simulink model "EDF"  (R2025b)
settings: Solver=VariableStepAuto  StartTime=0.0  StopTime=30  FixedStep=0.1  RelTol=1e-3
libraries: simulink x1, slpidlib x1
settings Model: Creator=wangzerun  LastModifiedBy=wangzerun

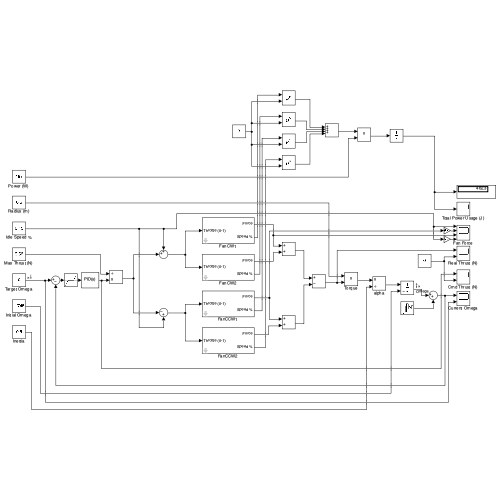
[thumbnail: Simulink's stored preview of the top-level diagram]
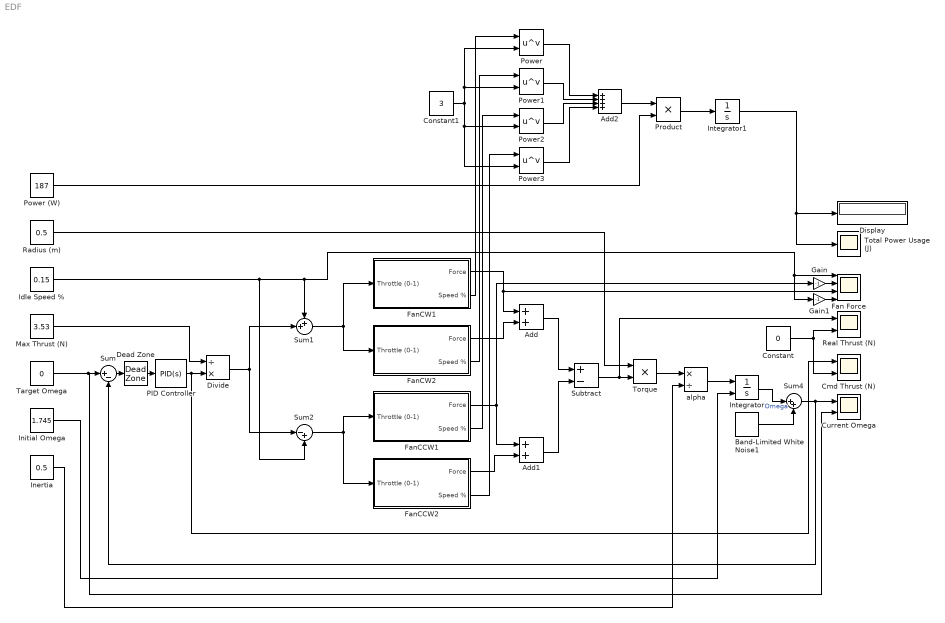
== system EDF ==
  Add : Sum
  Add1 : Sum
  Add2 : Sum  Inputs=++++
  Band-Limited White Noise1 : simulink/Sources/Band-Limited White Noise  Cov=(30 * pi/180)^2 * 2  Ts=2  seed=[23341]
  Cmd Thrust (N) : Scope  NumInputPorts=2
      settings: ActiveDisplayYMinimum=-12.321116744675173  ActiveDisplayYMaximum=4.742010611975001  DataLoggingVariableName=ScopeData3
  Constant : Constant  Value=0
  Constant1 : Constant  Value=3
  Current Omega : Scope  NumInputPorts=2
      settings: ActiveDisplayYMinimum=-4.3264371148966774  ActiveDisplayYMaximum=4.7874283495115693
  Dead Zone : DeadZone  LowerValue=-0.015  UpperValue=0.015
  Display : Display
  Divide : Product  Inputs=/*
  Fan Force : Scope  NumInputPorts=4
      settings: ActiveDisplayYMinimum=-5.5903004683370039  ActiveDisplayYMaximum=5.6346908697833626  DataLoggingVariableName=ScopeData4
  FanCCW1 : Subsystem  mask{tau=0.1, F_max=3.53}
      mask prompts: tau "Time Constant (s)"; F_max "Max Thrust (N)"
  FanCCW2 : Subsystem  mask{tau=0.15, F_max=3.53}
      mask prompts: tau "Time Constant (s)"; F_max "Max Thrust (N)"
  FanCW1 : Subsystem  mask{tau=0.1, F_max=3.53}
      mask prompts: tau "Time Constant (s)"; F_max "Max Thrust (N)"
  FanCW2 : Subsystem  mask{tau=0.1, F_max=3.53}
      mask prompts: tau "Time Constant (s)"; F_max "Max Thrust (N)"
  Gain : Gain  Gain=-1
  Gain1 : Gain  Gain=-1
  Idle Speed % : Constant  Value=0.15
  Inertia : Constant  Value=0.5
  Initial Omega : Constant  Value=1.745
  Integrator : Integrator  InitialConditionSource=external  InitialCondition=10
  Integrator1 : Integrator
  Max Thrust (N) : Constant  Value=3.53
  PID Controller : slpidlib/PID Controller  Controller=PID  Form=Parallel  TimeDomain=Continuous-time  UseExternalTs=off  SampleTime=0.1  IntegratorMethod=Forward Euler  FilterMethod=Forward Euler  ControllerParametersSource=internal  P=2.5  I=1  UseKiTs=off  D=4  UseExternalDerivativeSource=off  N=2  UseFilter=on  TunerSelectOption=Transfer Function Based (PID Tuner App)  InitialConditionSource=internal  InitialConditionForIntegrator=0  InitialConditionForFilter=0  DifferentiatorICPrevScaledInput=0  ExternalReset=none  TrackingMode=off  Kt=1  LimitOutput=off  SatLimitsSource=internal  UpperSaturationLimit=inf  LowerSaturationLimit=-inf  LinearizeAsGain=on  AntiWindupMode=none  Kb=1  LimitIntegrator=off  UpperIntegratorSaturationLimit=inf  LowerIntegratorSaturationLimit=-inf  POutMin=[]  POutMax=[]  IOutMin=[]  IOutMax=[]  DOutMin=[]  DOutMax=[]  NOutMin=[]  NOutMax=[]  SumOutMin=[]  SumOutMax=[]  SaturationOutMin=[]  SaturationOutMax=[]  PParamMin=[]  PParamMax=[]  IParamMin=[]  IParamMax=[]  DParamMin=[]  DParamMax=[]  NParamMin=[]  NParamMax=[]  KbParamMin=[]  KbParamMax=[]  KtParamMin=[]  KtParamMax=[]  KbOutMin=[]  KbOutMax=[]  KtOutMin=[]  KtOutMax=[]  IntegratorOutMin=[]  IntegratorOutMax=[]  FilterOutMin=[]  FilterOutMax=[]  SumI1OutMin=[]  SumI1OutMax=[]  SumI2OutMin=[]  SumI2OutMax=[]  SumI3OutMin=[]  SumI3OutMax=[]  SumI4OutMin=[]  SumI4OutMax=[]  SumDOutMin=[]  SumDOutMax=[]  DifferentiatorOutMin=[]  DifferentiatorOutMax=[]  FilterDiffOutCoefMin=[]  FilterDiffOutCoefMax=[]  ReciprocalOutMin=[]  ReciprocalOutMax=[]  SumDenOutMin=[]  SumDenOutMax=[]  SumNumOutMin=[]  SumNumOutMax=[]  DivideOutMin=[]  DivideOutMax=[]  UdiffTsProdOutMin=[]  UdiffTsProdOutMax=[]  NTsProdOutMin=[]  NTsProdOutMax=[]  UintegralTsProdOutMin=[]  UintegralTsProdOutMax=[]  UngainTsProdOutMin=[]  UngainTsProdOutMax=[]  ClampingZeroOutDataTypeStr=Inherit: Inherit via back propagation  ClampingZeroOutMin=[]  ClampingZeroOutMax=[]  FilterDenConstantOutDataTypeStr=Inherit: Inherit via back propagation  FilterDenConstantOutMin=[]  FilterDenConstantOutMax=[]  PCopyOutDataTypeStr=Inherit: Inherit via back propagation  PCopyOutMin=[]  PCopyOutMax=[]  NCopyOutDataTypeStr=Inherit: Inherit via back propagation  NCopyOutMin=[]  NCopyOutMax=[]  IntegratorContinuousStateAttributes=''  IntegratorStateMustResolveToSignalObject=off  IntegratorRTWStateStorageClass=Auto  FilterContinuousStateAttributes=''  FilterStateMustResolveToSignalObject=off  FilterRTWStateStorageClass=Auto  ParallelPVariant=InternalParameters  IdealPVariant=Disabled  IVariant=InternalParameters  DVariant=InternalParameters  IntegratorVariant=Continuous  SatVariant=Disabled  AWVariant=Passthrough  PCopyVariant=Disabled  TRVariant=Disabled  FdbkBlocksVariant=Forward  IdealPFdbkVariant=Disabled  SatFdbkVariant=Disabled  DerivativeFilterVariant=ContFilter  NVariant=InternalParameters  NCopyVariant=Disabled  FilterICVariant=InternalICsFilter  IntegratorICVariant=InternalICs  ExternalResetVariant=Disabled  TRSumVariant=Passthrough  SumFdbkVariant=Disabled  SumVariant=Sum_PID  TsampFilterVariant=InternalTs  TsampNgainVariant=Passthrough  TsampIntegralVariant=Disabled_SignalSpec  ExternalSaturationOutDataTypeStr=Inherit: Same as second input  DerivativeSourceVariant=ErrorSignal  PreIntVariant=InternalPreInt
  Power{,1..3} (4 alike) : Math  Operator=pow
  Power (W) : Constant  Value=187
  Product : Product
  Radius (m) : Constant  Value=0.5
  Real Thrust (N) : Scope  NumInputPorts=2
      settings: ActiveDisplayYMinimum=-2.9911384898343907  ActiveDisplayYMaximum=2.9859087354842568  DataLoggingVariableName=ScopeData2
  Subtract : Sum  Inputs=+-
  Sum : Sum  Inputs=|+-
  Sum1 : Sum  Inputs=++|
  Sum2 : Sum  Inputs=|-+
  Sum4 : Sum  Inputs=|++
  Target Omega : Constant  Value=0
  Torque : Product
  Total Power Usage (J) : Scope
      settings: ActiveDisplayYMinimum=-11.918034188673857  ActiveDisplayYMaximum=281.40339603355426
  alpha : Product  Inputs=*/
  wires:
  Target Omega/1 -> Current Omega/2, Sum/1
  Initial Omega/1 -> Integrator/2
  alpha/1 -> Integrator/1
  Inertia/1 -> alpha/2
  PID Controller/1 -> Cmd Thrust (N)/1, Divide/2
  Constant/1 -> Cmd Thrust (N)/2, Real Thrust (N)/2
  Max Thrust (N)/1 -> Divide/1
  Idle Speed %/1 -> Sum2/2, Gain1/1, Fan Force/1, Sum1/1
  Divide/1 -> Sum2/1, Sum1/2
  Sum1/1 -> FanCW2/1(Throttle (0-1)), FanCW1/1(Throttle (0-1))
  Sum2/1 -> FanCCW2/1(Throttle (0-1)), FanCCW1/1(Throttle (0-1))
  FanCW1/1(Force) -> Fan Force/3, Add/1
  FanCW2/1(Force) -> Add/2
  FanCCW1/1(Force) -> Add1/1, Gain/1
  FanCCW2/1(Force) -> Add1/2
  Add1/1 -> Subtract/2
  Add/1 -> Subtract/1
  Subtract/1 -> Real Thrust (N)/1, Torque/2
  Radius (m)/1 -> Torque/1
  Torque/1 -> alpha/1
  Gain/1 -> Fan Force/2
  Gain1/1 -> Fan Force/4
  FanCW1/2(Speed %) -> Power/1
  FanCW2/2(Speed %) -> Power1/1
  FanCCW1/2(Speed %) -> Power2/1
  FanCCW2/2(Speed %) -> Power3/1
  Constant1/1 -> Power2/2, Power3/2, Power1/2, Power/2
  Power/1 -> Add2/1
  Power1/1 -> Add2/2
  Power2/1 -> Add2/3
  Power3/1 -> Add2/4
  Add2/1 -> Product/1
  Power (W)/1 -> Product/2
  Product/1 -> Integrator1/1
  Integrator1/1 -> Display/1, Total Power Usage (J)/1
  Integrator/1 -> Sum4/1  "Omega"
  Band-Limited White Noise1/1 -> Sum4/2
  Sum4/1 -> Sum/2, Current Omega/1
  Sum/1 -> Dead Zone/1
  Dead Zone/1 -> PID Controller/1

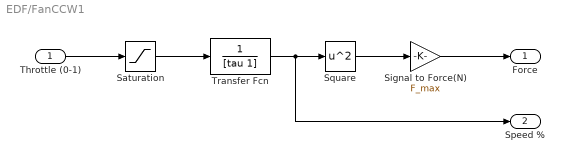
== system EDF/FanCCW1 ==
  Throttle (0-1) : Inport
  Saturation : Saturate  UpperLimit=1  LowerLimit=0.1
  Signal to Force(N) : Gain  Gain=F_max
  Square : Math  Operator=square
  Transfer Fcn : TransferFcn  Denominator=[tau 1]
  Force : Outport
  Speed % : Outport  Port=2
  wires:
  Saturation/1 -> Transfer Fcn/1
  Square/1 -> Signal to Force(N)/1
  Transfer Fcn/1 -> Speed %/1, Square/1
  Throttle (0-1)/1 -> Saturation/1
  Signal to Force(N)/1 -> Force/1

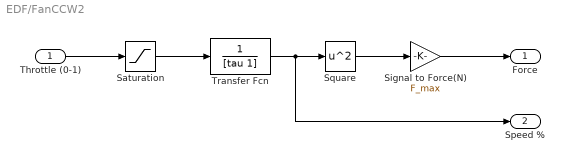
== system EDF/FanCCW2 ==
  Throttle (0-1) : Inport
  Saturation : Saturate  UpperLimit=1  LowerLimit=0.1
  Signal to Force(N) : Gain  Gain=F_max
  Square : Math  Operator=square
  Transfer Fcn : TransferFcn  Denominator=[tau 1]
  Force : Outport
  Speed % : Outport  Port=2
  wires:
  Saturation/1 -> Transfer Fcn/1
  Square/1 -> Signal to Force(N)/1
  Transfer Fcn/1 -> Speed %/1, Square/1
  Throttle (0-1)/1 -> Saturation/1
  Signal to Force(N)/1 -> Force/1

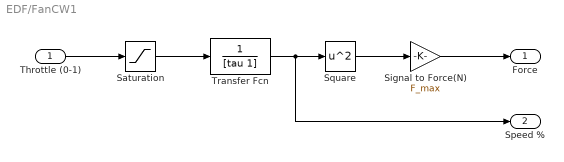
== system EDF/FanCW1 ==
  Throttle (0-1) : Inport
  Saturation : Saturate  UpperLimit=1  LowerLimit=0.1
  Signal to Force(N) : Gain  Gain=F_max
  Square : Math  Operator=square
  Transfer Fcn : TransferFcn  Denominator=[tau 1]
  Force : Outport
  Speed % : Outport  Port=2
  wires:
  Saturation/1 -> Transfer Fcn/1
  Square/1 -> Signal to Force(N)/1
  Transfer Fcn/1 -> Speed %/1, Square/1
  Throttle (0-1)/1 -> Saturation/1
  Signal to Force(N)/1 -> Force/1

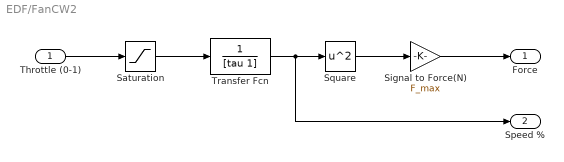
== system EDF/FanCW2 ==
  Throttle (0-1) : Inport
  Saturation : Saturate  UpperLimit=1  LowerLimit=0.1
  Signal to Force(N) : Gain  Gain=F_max
  Square : Math  Operator=square
  Transfer Fcn : TransferFcn  Denominator=[tau 1]
  Force : Outport
  Speed % : Outport  Port=2
  wires:
  Saturation/1 -> Transfer Fcn/1
  Square/1 -> Signal to Force(N)/1
  Transfer Fcn/1 -> Speed %/1, Square/1
  Throttle (0-1)/1 -> Saturation/1
  Signal to Force(N)/1 -> Force/1
